simulink model "force_position_step3_3"  (R2025b)
settings: Solver=VariableStepAuto  StartTime=0.0  StopTime=1  RelTol=1e-3
values from neighbouring files (symbols this model uses):
  lut_i_mA = interp1(z_anchor_um, i_anchor_mA, lut_z_um, 'pchip')    [init_force_position_sim_step2.m]
  lut_z_um = linspace(min(z_anchor_um), max(z_anchor_um), 501)    [init_force_position_sim_step2.m]
settings Model: Creator=HYB  LastModifiedBy=HYB

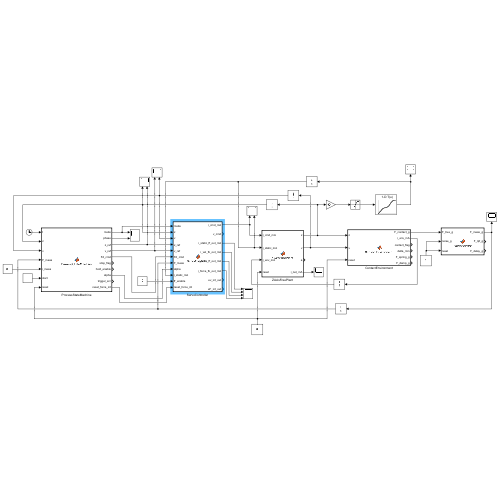
[thumbnail: Simulink's stored preview of the top-level diagram]
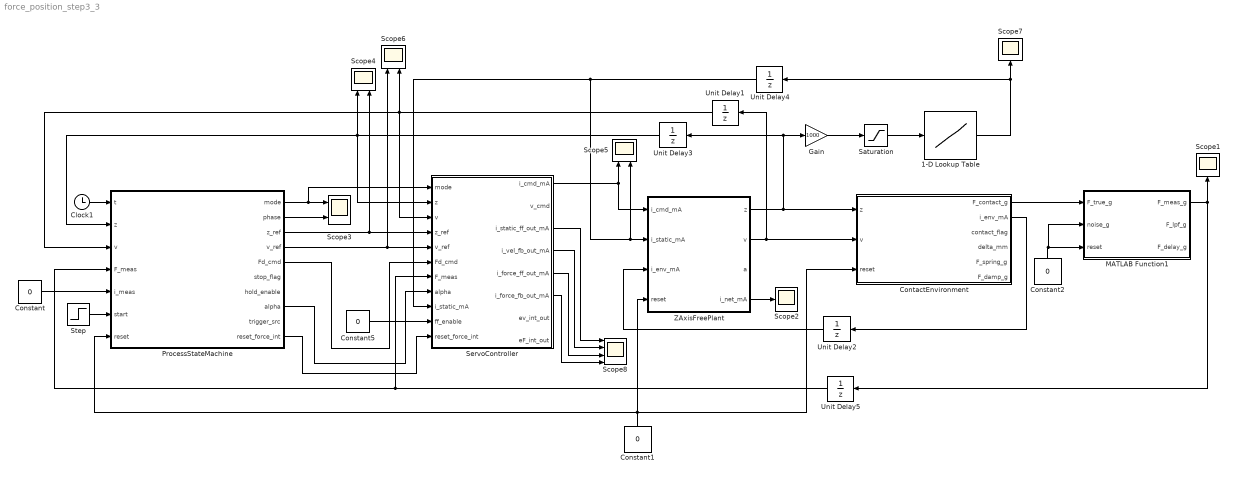
== system force_position_step3_3 ==
  1-D Lookup Table : Lookup_n-D  NumberOfTableDimensions=1  BreakpointsForDimension1=lut_z_um  Table=lut_i_mA  InternalRulePriority=Speed  RndMeth=Simplest
  Clock1 : Clock
  Constant{,1..2,5} (4 alike) : Constant  Value=0
  ContactEnvironment : MATLAB Function  TreatAsAtomicUnit=on
  Gain : Gain  Gain=1000
  MATLAB Function1 : MATLAB Function  TreatAsAtomicUnit=on
  ProcessStateMachine : MATLAB Function  TreatAsAtomicUnit=on
  Saturation : Saturate  UpperLimit=15000  LowerLimit=0
  Scope1 : Scope
      settings: ActiveDisplayYMinimum=-186.81719571271276  ActiveDisplayYMaximum=1681.3547614144152
  Scope2 : Scope
      settings: ActiveDisplayYMinimum=-1967.6933461484089  ActiveDisplayYMaximum=1895.5357153815362
  Scope{3..6} (4 alike) : Scope  NumInputPorts=2
      Scope3 settings: ActiveDisplayYMinimum=-0.49999999999999989  ActiveDisplayYMaximum=4.5  DataLoggingVariableName=ScopeData3
      Scope4 settings: ActiveDisplayYMinimum=12.909563525543636  ActiveDisplayYMaximum=15.227705203289965  DataLoggingVariableName=ScopeData4
      Scope5 settings: ActiveDisplayYMinimum=-403.88890728908666  ActiveDisplayYMaximum=1479.7302904427656  DataLoggingVariableName=ScopeData5
      Scope6 settings: ActiveDisplayYMinimum=-1.7987178186952431  ActiveDisplayYMaximum=12.161900299919697  DataLoggingVariableName=ScopeData6
  Scope7 : Scope
      settings: ActiveDisplayYMinimum=800.135408652136  ActiveDisplayYMaximum=882.66437213169263  DataLoggingVariableName=ScopeData7
  Scope8 : Scope  NumInputPorts=4
      settings: ActiveDisplayYMinimum=-685.21477393206442  ActiveDisplayYMaximum=1959.6446227297147  DataLoggingVariableName=ScopeData2
  ServoController : MATLAB Function  TreatAsAtomicUnit=on
  Step : Step  Time=0.01  SampleTime=0
  Unit Delay{1..5} (5 alike) : UnitDelay  SampleTime=0.001  HasFrameUpgradeWarning=on
  ZAxisFreePlant : MATLAB Function  TreatAsAtomicUnit=on
  wires:
  ServoController/6(i_force_fb_out_mA) -> Scope8/4
  Constant5/1 -> ServoController/10(ff_enable)
  ContactEnvironment/2(i_env_mA) -> Unit Delay2/1
  Unit Delay1/1 -> ServoController/3(v), ProcessStateMachine/3(v), Scope6/2
  ServoController/3(i_static_ff_out_mA) -> Scope8/1
  ContactEnvironment/1(F_contact_g) -> MATLAB Function1/1(F_true_g)
  ProcessStateMachine/5(Fd_cmd) -> ServoController/6(Fd_cmd)
  Saturation/1 -> 1-D Lookup Table/1
  ZAxisFreePlant/1(z) -> ContactEnvironment/1(z), Unit Delay3/1, Gain/1
  Gain/1 -> Saturation/1
  ZAxisFreePlant/4(i_net_mA) -> Scope2/1
  Unit Delay2/1 -> ZAxisFreePlant/3(i_env_mA)
  Step/1 -> ProcessStateMachine/6(start)
  ZAxisFreePlant/2(v) -> ContactEnvironment/2(v), Unit Delay1/1
  ServoController/5(i_force_ff_out_mA) -> Scope8/3
  ProcessStateMachine/1(mode) -> Scope3/1, ServoController/1(mode)
  Clock1/1 -> ProcessStateMachine/1(t)
  ProcessStateMachine/3(z_ref) -> ServoController/4(z_ref), Scope4/2
  ProcessStateMachine/10(reset_force_int) -> ServoController/11(reset_force_int)
  ServoController/4(i_vel_fb_out_mA) -> Scope8/2
  ServoController/1(i_cmd_mA) -> ZAxisFreePlant/1(i_cmd_mA), Scope5/1
  Unit Delay5/1 -> ProcessStateMachine/4(F_meas), ServoController/7(F_meas)
  1-D Lookup Table/1 -> Unit Delay4/1, Scope7/1
  Constant/1 -> ProcessStateMachine/5(i_meas)
  Unit Delay3/1 -> ServoController/2(z), ProcessStateMachine/2(z), Scope4/1
  ProcessStateMachine/4(v_ref) -> ServoController/5(v_ref), Scope6/1
  ProcessStateMachine/8(alpha) -> ServoController/8(alpha)
  Unit Delay4/1 -> Scope5/2, ZAxisFreePlant/2(i_static_mA), ServoController/9(i_static_mA)
  Constant1/1 -> ContactEnvironment/3(reset), ZAxisFreePlant/4(reset), ProcessStateMachine/7(reset)
  ProcessStateMachine/2(phase) -> Scope3/2
  MATLAB Function1/1(F_meas_g) -> Unit Delay5/1, Scope1/1
  Constant2/1 -> MATLAB Function1/2(noise_g), MATLAB Function1/3(reset)

== matlab function force_position_step3_3/ZAxisFreePlant ==
  data: i_cmd_mA input; z output; i_static_mA input; i_env_mA input; reset input; v output; a output; i_net_mA output
function [z, v, a, i_net_mA] = ZAxisFreePlant(i_cmd_mA, i_static_mA, i_env_mA, reset)
%#codegen

% ============================================================
% 简化Z轴自由运动模型
%
% 下行方向为正：
%   z 增大表示压头向下伸出
%
% i_static_mA 是实验一得到的下行静态保持电流。
% 在对象模型中，它作为位置相关的非线性负载项。
%
% 简化模型：
%   a = Kacc * (i_cmd - i_static(z) - Cv*v - Icoul*tanh(v/vs))
% ============================================================

%% 参数
Ts = 1e-3;

z0 = 0.0;          % 初始位置，mm
v0 = 0.0;

z_min = 0.0;
z_max = 15.2;      % 比实际15mm略大一点，便于保护观察

Kacc = 20.0;        % mm/s^2 per mA
Cv_mA = 1.0;       % mA/(mm/s)
Icoul_mA = 2.0;    % mA
vs = 0.05;         % mm/s，tanh平滑速度

persistent z_k v_k

if isempty(z_k)
    z_k = z0;
    v_k = v0;
end

if reset
    z_k = z0;
    v_k = v0;
end

%% 摩擦电流
i_fric_mA = Cv_mA * v_k + Icoul_mA * tanh(v_k / vs);

%% 净驱动电流
i_net_mA = i_cmd_mA - i_static_mA - i_fric_mA - i_env_mA;

%% 加速度
a = Kacc * i_net_mA;

%% 积分
v_k = v_k + Ts * a;
z_k = z_k + Ts * v_k;

%% 行程限位
if z_k < z_min
    z_k = z_min;
    if v_k < 0
        v_k = 0.0;
    end
elseif z_k > z_max
    z_k = z_max;
    if v_k > 0
        v_k = 0.0;
    end
end

z = z_k;
v = v_k;

== matlab function force_position_step3_3/ServoController ==
  data: mode input; i_cmd_mA output; z input; v input; z_ref input; v_ref input; Fd_cmd input; F_meas input; alpha input; i_static_mA input; ff_enable input; reset_force_int input; v_cmd output; i_static_ff_out_mA output; i_vel_fb_out_mA output; i_force_ff_out_mA output; i_force_fb_out_mA output; ev_int_out output; eF_int_out output
function [i_cmd_mA, v_cmd, i_static_ff_out_mA, i_vel_fb_out_mA, ...
          i_force_ff_out_mA, i_force_fb_out_mA, ev_int_out, eF_int_out] = ...
    ServoController(mode, z, v, z_ref, v_ref, Fd_cmd, F_meas, alpha, ...
                    i_static_mA, ff_enable, reset_force_int)
%#codegen

% ============================================================
% ServoController
%
% 功能：
%   mode = 1：位置模式
%       位置误差 -> 速度指令 -> 速度PI -> 电流
%
%   mode = 2：速度模式
%       速度指令 -> 速度PI -> 电流
%
%   mode = 3：力矩/电流保压模式
%       静态前馈 + 目标力前馈 + 力反馈
%       注意：此时不再使用速度PI，否则就不是力矩模式
%
%   mode = 9：安全停止
%
% 输入：
%   mode            : 控制模式
%   z               : 当前位移，mm，下行为正
%   v               : 当前速度，mm/s，下行为正
%   z_ref           : 位置目标，mm
%   v_ref           : 速度目标，mm/s
%   Fd_cmd          : 目标力，g
%   F_meas          : 测得接触力，g
%   alpha           : 力前馈平滑引入系数，0~1
%   i_static_mA     : 静态位置补偿电流，mA
%   ff_enable       : 静态前馈开关，1开启，0关闭
%   reset_force_int : 进入保压时复位力积分
%
% 输出：
%   i_cmd_mA          : 最终电流指令，mA
%   v_cmd             : 控制器内部速度指令，mm/s
%   i_static_ff_out_mA: 静态前馈电流，mA
%   i_vel_fb_out_mA   : 速度环反馈电流，mA
%   i_force_ff_out_mA : 目标力前馈电流，mA
%   i_force_fb_out_mA : 力反馈电流，mA
%   ev_int_out        : 速度积分状态
%   eF_int_out        : 力积分状态
% ============================================================

%% ============================================================
% 1. 基本参数
% ============================================================

Ts = 1e-3;              % 控制周期，s

%% 位置环参数
Kp_pos = 100.0;         % 位置环比例，输出速度，(mm/s)/mm
v_fast_max = 100.0;     % 位置模式最大速度，mm/s

%% 速度PI参数
Kvp = 20.0;             % 速度比例增益，mA/(mm/s)
Kvi = 200.0;            % 速度积分增益，mA/(mm)

i_vel_int_limit = 3000.0;   % 速度积分电流限幅，mA

%% 力前馈与力反馈参数
% 这里先认为 1 g 对应 1 mA。
% 后续如果实测 200 mA 不等于 200 g，需要重新标定这个系数。
Kforce_mA_per_g = 1.0;      % 力前馈系数，mA/g

% 第一版建议先用很小的力反馈，避免接触模型刚接入时振荡
force_fb_enable = 1.0;      % 1 开启力反馈；0 只用力前馈

Kpf = 0.5;                  % 力反馈比例，mA/g
Kif = 5;                 % 力反馈积分，mA/(g*s)

i_force_int_limit = 1000.0; % 力积分电流限幅，mA

%% 总电流限幅
i_limit = 5000.0;           % 电流峰值限制，mA，即 5A

%% ============================================================
% 2. 持久变量
% ============================================================

persistent ev_int eF_int last_mode

if isempty(ev_int)
    ev_int = 0.0;
    eF_int = 0.0;
    last_mode = 0.0;
end

%% ============================================================
% 3. 模式切换处理
% ============================================================

% 进入力矩/保压模式时，复位力积分
if reset_force_int
    eF_int = 0.0;
end

% 从速度/位置模式切到力矩模式时，清掉速度积分
% 防止前一阶段速度环积分残留影响后续判断
if last_mode ~= 3 && mode == 3
    ev_int = 0.0;
end

% 进入安全停止时，清空积分
if mode == 9
    ev_int = 0.0;
    eF_int = 0.0;
end

%% ============================================================
% 4. 默认输出初始化
% ============================================================

v_cmd = 0.0;

i_static_ff_mA = 0.0;
i_vel_fb_mA = 0.0;
i_force_ff_mA = 0.0;
i_force_fb_mA = 0.0;

%% ============================================================
% 5. 静态前馈
% ============================================================

if ff_enable > 0.5
    i_static_ff_mA = i_static_mA;
else
    i_static_ff_mA = 0.0;
end

%% ============================================================
% 6. 不同模式下的控制律
% ============================================================

if mode == 1
    %% --------------------------------------------------------
    % 位置模式：位置外环 + 速度PI
    % ---------------------------------------------------------
    
    e_pos = z_ref - z;
    v_cmd = Kp_pos * e_pos;
    
    % 速度限幅
    if v_cmd > v_fast_max
        v_cmd = v_fast_max;
    elseif v_cmd < -v_fast_max
        v_cmd = -v_fast_max;
    end
    
    % 速度PI
    e_v = v_cmd - v;
    
    i_v_p = Kvp * e_v;
    
    ev_int = ev_int + e_v * Ts;
    i_v_i = Kvi * ev_int;
    
    % 速度积分限幅
    if i_v_i > i_vel_int_limit
        i_v_i = i_vel_int_limit;
        ev_int = i_v_i / Kvi;
    elseif i_v_i < -i_vel_int_limit
        i_v_i = -i_vel_int_limit;
        ev_int = i_v_i / Kvi;
    end
    
    i_vel_fb_mA = i_v_p + i_v_i;
    
elseif mode == 2
    %% --------------------------------------------------------
    % 速度模式：速度PI
    % ---------------------------------------------------------
    
    v_cmd = v_ref;
    
    e_v = v_cmd - v;
    
    i_v_p = Kvp * e_v;
    
    ev_int = ev_int + e_v * Ts;
    i_v_i = Kvi * ev_int;
    
    % 速度积分限幅
    if i_v_i > i_vel_int_limit
        i_v_i = i_vel_int_limit;
        ev_int = i_v_i / Kvi;
    elseif i_v_i < -i_vel_int_limit
        i_v_i = -i_vel_int_limit;
        ev_int = i_v_i / Kvi;
    end
    
    i_vel_fb_mA = i_v_p + i_v_i;
    
elseif mode == 3
    %% --------------------------------------------------------
    % 力矩/电流保压模式
    %
    % 注意：
    %   这里不再使用速度PI。
    %   电流由：
    %       静态前馈 + 目标力前馈 + 力反馈
    %   组成。
    % ---------------------------------------------------------
    
    v_cmd = 0.0;
    
    % 目标力前馈，alpha由状态机给出，0 -> 1 平滑引入
    i_force_ff_mA = alpha * Kforce_mA_per_g * Fd_cmd;
    
    % 力反馈
    if force_fb_enable > 0.5
        eF = Fd_cmd - F_meas;
        
        eF_int = eF_int + eF * Ts;
        iF_i = Kif * eF_int;
        
        % 力积分限幅
        if iF_i > i_force_int_limit
            iF_i = i_force_int_limit;
            eF_int = iF_i / Kif;
        elseif iF_i < -i_force_int_limit
            iF_i = -i_force_int_limit;
            eF_int = iF_i / Kif;
        end
        
        iF_p = Kpf * eF;
        
        i_force_fb_mA = iF_p + iF_i;
    else
        i_force_fb_mA = 0.0;
    end
    
    % 保压模式下速度环关闭
    i_vel_fb_mA = 0.0;
    
elseif mode == 9
    %% --------------------------------------------------------
    % 安全停止
    % ---------------------------------------------------------
    
    v_cmd = 0.0;
    
    i_static_ff_mA = 0.0;
    i_vel_fb_mA = 0.0;
    i_force_ff_mA = 0.0;
    i_force_fb_mA = 0.0;
    
else
    %% --------------------------------------------------------
    % Ready / Off
    % ---------------------------------------------------------
    
    v_cmd = 0.0;
    
    i_static_ff_mA = 0.0;
    i_vel_fb_mA = 0.0;
    i_force_ff_mA = 0.0;
    i_force_fb_mA = 0.0;
end

%% ============================================================
% 7. 合成电流
% ============================================================

i_cmd_unsat = i_static_ff_mA ...
            + i_vel_fb_mA ...
            + i_force_ff_mA ...
            + i_force_fb_mA;

i_cmd_mA = i_cmd_unsat;

%% 总电流限幅
if i_cmd_mA > i_limit
    i_cmd_mA = i_limit;
elseif i_cmd_mA < -i_limit
    i_cmd_mA = -i_limit;
end

%% ============================================================
% 8. 简单抗积分饱和
% ============================================================

% 如果速度/位置模式下总电流饱和，且速度积分还在推动饱和方向，
% 则回退一部分速度积分。
if mode == 1 || mode == 2
    if i_cmd_unsat ~= i_cmd_mA
        e_v_aw = v_cmd - v;
        
        if (i_cmd_unsat > i_limit && e_v_aw > 0.0) || ...
           (i_cmd_unsat < -i_limit && e_v_aw < 0.0)
            ev_int = ev_int - 0.5 * e_v_aw * Ts;
        end
    end
end

% 如果力矩模式下总电流饱和，且力积分还在推动饱和方向，
% 则回退一部分力积分。
if mode == 3 && force_fb_enable > 0.5
    if i_cmd_unsat ~= i_cmd_mA
        eF_aw = Fd_cmd - F_meas;
        
        if (i_cmd_unsat > i_limit && eF_aw > 0.0) || ...
           (i_cmd_unsat < -i_limit && eF_aw < 0.0)
            eF_int = eF_int - 0.5 * eF_aw * Ts;
        end
    end
end

%% ============================================================
% 9. 输出监控量
% ============================================================

i_static_ff_out_mA = i_static_ff_mA;
i_vel_fb_out_mA    = i_vel_fb_mA;
i_force_ff_out_mA  = i_force_ff_mA;
i_force_fb_out_mA  = i_force_fb_mA;

ev_int_out = ev_int;
eF_int_out = eF_int;

last_mode = mode;

== matlab function force_position_step3_3/ProcessStateMachine ==
  data: t input; mode output; z input; v input; F_meas input; i_meas input; start input; reset input; phase output; z_ref output; v_ref output; Fd_cmd output; stop_flag output; hold_enable output; alpha output; trigger_src output; reset_force_int output
function [mode, phase, z_ref, v_ref, Fd_cmd, stop_flag, hold_enable, alpha, trigger_src, reset_force_int] = ...
    ProcessStateMachine(t, z, v, F_meas, i_meas, start, reset)
%#codegen

% ============================================================
% 力位控制工艺流程状态机
% 阶段：
% 0 Ready
% 1 FastPosition: 位置模式快进到 13 mm
% 2 FirstVelocity: 第一速度到 14 mm
% 3 SearchVelocity: 第二速度搜索接触
% 4 ForceHold: 力矩/电流模式保压
% 5 ErrorStop: 超行程或异常停止
% ============================================================


%% ---------- 可调参数 ----------
z_fast_end = 13.0;     % mm
z_v1_end   = 14.0;     % mm
z_max      = 15.0;     % mm

pos_tol = 0.02;        % mm

v1_search = 5.0;       % mm/s
v2_search = 1.0;       % mm/s

F_th = 10.0;           % g
T_force_confirm = 0.001;   % s

v_stop_th = 0.05;          % mm/s
T_v_confirm = 0.005;       % s

% 第一版暂不启用电流判断，所以阈值给很大
i_stop_th = 1e9;
T_i_confirm = 0.003;       % s

Fd_set = 1000.0;            % g
T_ramp_force = 0.010;      % s

%% ---------- 状态变量 ----------
persistent state t_enter tF_start tV_start tI_start prev_state

if isempty(state)
    state = int32(0);
    prev_state = int32(0);
    t_enter = 0.0;
    tF_start = -1.0;
    tV_start = -1.0;
    tI_start = -1.0;
end

if reset
    state = int32(0);
    prev_state = int32(0);
    t_enter = t;
    tF_start = -1.0;
    tV_start = -1.0;
    tI_start = -1.0;
end

%% ---------- 默认输出 ----------
mode = 0;
phase = double(state);
z_ref = z; % 默认保持住位置，防止突然运动
v_ref = 0.0;
Fd_cmd = Fd_set; % 默认力指令就设置为力设定值，切换为力控时目标力则已经是设定值
stop_flag = false; % 默认不停止，运行外部控制器继续执行位置/速度环
hold_enable = false; % 默认禁用积分器保持，在状态4会开启，力控时造成的位移累积误差在切换回位控时可以快速恢复
alpha = 0.0; % 在状态4时会从0平滑过渡到1
trigger_src = 0;       % 0 none, 1 force, 2 velocity, 3 current, 4 z_max
reset_force_int = false; % 默认不复位力控积分器，只在进入状态4的瞬间设1

prev_state = state;

%% ---------- 启动逻辑 ----------
if state == 0
    mode = 0;
    phase = 0;
    z_ref = z;
    v_ref = 0.0;
    alpha = 0.0;
    
    if start % 一般阶跃输入
        state = int32(1);
        t_enter = t; % 进入当前状态的时间戳
    end
end

%% ---------- 状态 1：位置快进 ----------
if state == 1
    mode = 1;
    phase = 1;
    z_ref = z_fast_end;
    v_ref = 0.0;
    alpha = 0.0;
    
    if z >= z_fast_end - pos_tol
        state = int32(2);
        t_enter = t;
    end
end

%% ---------- 状态 2：第一速度 ----------
if state == 2
    mode = 2;          % 速度模式
    phase = 2;
    z_ref = z;
    v_ref = v1_search;
    alpha = 0.0;
    
    if z >= z_v1_end - pos_tol
        state = int32(3);
        t_enter = t;
        tF_start = -1.0;
        tV_start = -1.0;
        tI_start = -1.0;
    end
end

%% ---------- 状态 3：第二速度搜索 ----------
if state == 3
    mode = 2;          % 速度模式
    phase = 3;
    z_ref = z;
    v_ref = v2_search;
    alpha = 0.0;
    
    % --- 压力触发 ---
    if F_meas > F_th
        if tF_start < 0.0
            tF_start = t;
        end
    else
        tF_start = -1.0;
    end
    
    force_ok = false;
    if tF_start >= 0.0
        if (t - tF_start) >= T_force_confirm
            force_ok = true;
        end
    end
    
    % --- 速度触发，第一版作为备用 ---
    if abs(v) < v_stop_th
        if tV_start < 0.0
            tV_start = t;
        end
    else
        tV_start = -1.0;
    end
    
    velocity_ok = false;
    if tV_start >= 0.0
        if (t - tV_start) >= T_v_confirm
            velocity_ok = true;
        end
    end
    
    % --- 电流触发，第一版实际不会触发 ---
    if abs(i_meas) > i_stop_th
        if tI_start < 0.0
            tI_start = t;
        end
    else
        tI_start = -1.0;
    end
    
    current_ok = false;
    if tI_start >= 0.0
        if (t - tI_start) >= T_i_confirm
            current_ok = true;
        end
    end
    
    % --- 停止条件 ---
    if force_ok
        state = int32(4);
        t_enter = t;
        trigger_src = 1;
        stop_flag = true;
    elseif velocity_ok
        state = int32(4);
        t_enter = t;
        trigger_src = 2;
        stop_flag = true;
    elseif current_ok
        state = int32(4);
        t_enter = t;
        trigger_src = 3;
        stop_flag = true;
    elseif z >= z_max
        state = int32(5);
        t_enter = t;
        trigger_src = 4;
    end
end

%% ---------- 状态 4：力矩/电流模式保压 ----------
if state == 4
    mode = 3;          % 力矩/电流模式
    phase = 4;
    z_ref = z;
    v_ref = 0.0;
    Fd_cmd = Fd_set;
    stop_flag = true;
    hold_enable = true;
    
    % 目标力前馈平滑引入系数 alpha: 0 -> 1
    tau = (t - t_enter) / T_ramp_force;
    if tau < 0.0
        tau = 0.0;
    elseif tau > 1.0
        tau = 1.0;
    end
    
    % S型平滑
    alpha = 3.0*tau*tau - 2.0*tau*tau*tau;
end

%% ---------- 状态 5：安全停止 ----------
if state == 5
    mode = 9;
    phase = 5;
    z_ref = z;
    v_ref = 0.0;
    Fd_cmd = 0.0;
    stop_flag = true;
    hold_enable = false;
    alpha = 0.0;
end

%% ---------- 进入保压瞬间复位力控积分 ----------
if prev_state ~= int32(4) && state == int32(4)
    reset_force_int = true;
else
    reset_force_int = false;
end

phase = double(state);

== matlab function force_position_step3_3/ContactEnvironment ==
  data: z input; F_contact_g output; v input; reset input; i_env_mA output; contact_flag output; delta_mm output; F_spring_g output; F_damp_g output
function [F_contact_g, i_env_mA, contact_flag, delta_mm, F_spring_g, F_damp_g] = ContactEnvironment(z, v, reset)
%#codegen

z_contact = 14.30;       % mm

Ke_g_per_mm = 2000.0;    % g/mm
Be_g_per_mmps = 20.0;    % g/(mm/s)

F_max_g = 3000.0;
Kforce_mA_per_g = 1.0;

delta = z - z_contact;

if delta <= 0
    delta_mm = 0.0;
    F_spring_g = 0.0;
    F_damp_g = 0.0;
    F_contact_g = 0.0;
    contact_flag = false;
else
    delta_mm = delta;
    contact_flag = true;

    F_spring_g = Ke_g_per_mm * delta_mm;

    % 只在继续向下压入时产生正阻尼力
    if v > 0
        F_damp_g = Be_g_per_mmps * v;
    else
        F_damp_g = 0.0;
    end

    F_contact_g = F_spring_g + F_damp_g;

    if F_contact_g > F_max_g
        F_contact_g = F_max_g;
    end
end

i_env_mA = Kforce_mA_per_g * F_contact_g;

== matlab function force_position_step3_3/MATLAB Function1 ==
  data: F_true_g input; F_meas_g output; noise_g input; reset input; F_lpf_g output; F_delay_g output
function [F_meas_g, F_lpf_g, F_delay_g] = ForceSensor(F_true_g, noise_g, reset)
%#codegen

% ============================================================
% ForceSensor
%
% 作用：
%   将真实接触力 F_true_g 转换为控制器可见的测量力 F_meas_g。
%
% 模型包含：
%   1. 传感器量程限幅
%   2. 一阶低通滤波
%   3. 采样/传输延迟
%   4. 零偏和噪声
%
% 注意：
%   这个模块只用于测量反馈；
%   环境反力 i_env_mA 不应经过该模块再作用到 ZAxisFreePlant。
% ============================================================

%% 参数
Ts = 1e-3;              % s
tau_sensor = 0.005;     % s，传感器/滤波时间常数
F_sensor_max = 3000.0;  % g，传感器量程上限
F_sensor_min = 0.0;     % g，压缩力为正，第一版不考虑拉力

F_bias = 0.0;           % g，零偏

% 延迟采样点数
% 这里固定为 3，对应 3 ms
N_delay = 1;

%% 一阶低通系数
alpha = exp(-Ts / tau_sensor);

%% 持久变量
persistent y_lpf delay_buf initialized

if isempty(initialized)
    y_lpf = 0.0;
    delay_buf = zeros(1, N_delay);
    initialized = true;
end

if reset
    y_lpf = 0.0;
    delay_buf = zeros(1, N_delay);
end

%% 1. 量程限幅
F_sat = F_true_g;

if F_sat > F_sensor_max
    F_sat = F_sensor_max;
elseif F_sat < F_sensor_min
    F_sat = F_sensor_min;
end

%% 2. 一阶低通滤波
y_lpf = alpha * y_lpf + (1.0 - alpha) * F_sat;
F_lpf_g = y_lpf;

%% 3. 整数采样延迟
% delay_buf(1) 是最旧值，delay_buf(end) 是最新值
F_delay_g = delay_buf(1);

for k = 1:N_delay-1
    delay_buf(k) = delay_buf(k+1);
end
delay_buf(N_delay) = F_lpf_g;

%% 4. 加零偏和噪声
F_meas_g = F_delay_g + F_bias + noise_g;

%% 5. 测量值再次限幅
if F_meas_g > F_sensor_max
    F_meas_g = F_sensor_max;
elseif F_meas_g < F_sensor_min
    F_meas_g = F_sensor_min;
end
